simulink model "flightSimulation"  (R2026a)
settings: Solver=ode3  StartTime=0  StopTime=10  FixedStep=Ts  EnableMultiTasking=on
undefined symbols (not defined in the file or in its folder): ft, initPosSim3d, m, s, Ts
libraries: aerolibconvert2 x4, aerolibanimutils x2, environmentLibrary x2, sensorsLibrary x2, aerolibfltsims x2, aerolibsim3d x2, SignalEditorBlockLib x1, sim3dlib x1
settings Model: Creator=The MathWorks, Inc.  LastModifiedBy=The MathWorks, Inc.
settings OptimizationCC: BufferReuse=off
settings DebuggingCC: UnderspecifiedInitializationDetection=Classic  PregeneratedLibrarySubsystemCodeDiagnostic=none
settings HardwareCC: ProdHWDeviceType=32-bit Generic

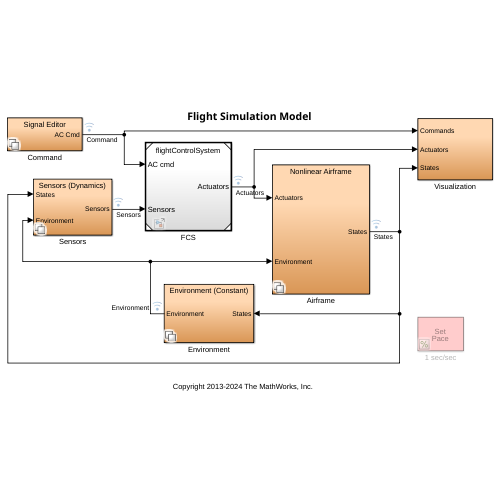
[thumbnail: Simulink's stored preview of the top-level diagram]
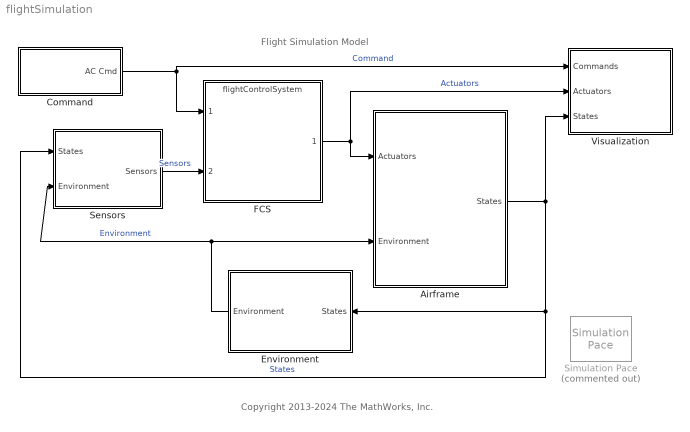
== system flightSimulation ==
  note: Flight Simulation Model
  note: Copyright 2013-2024 The MathWorks, Inc.
  Airframe : Subsystem  Variant=on
  Command : Subsystem  Variant=on
  Environment : Subsystem  Variant=on
  FCS : ModelReference  ModelNameDialog=flightControlSystem.slx  SimulationMode=Normal  ModelReferenceVersion=13.0
  Sensors : Subsystem  Variant=on
  Simulation Pace : aerolibanimutils/Simulation Pace  Commented=on  SimulationPace=1  SleepMode=MATLAB Thread  OutputPaceError=off  SampleTime=Ts
      settings: AttributesFormatString=%<SimulationPace> sec/sec
  Visualization : Subsystem
  wires:
  Command/1(AC Cmd) -> Visualization/1(Commands), FCS/1  "Command"
  Sensors/1(Sensors) -> FCS/2  "Sensors"
  FCS/1 -> Visualization/2(Actuators), Airframe/1(Actuators)  "Actuators"
  Environment/1(Environment) -> Sensors/2(Environment), Airframe/2(Environment)  "Environment"
  Airframe/1(States) -> Visualization/3(States), Environment/1(States), Sensors/1(States)  "States"

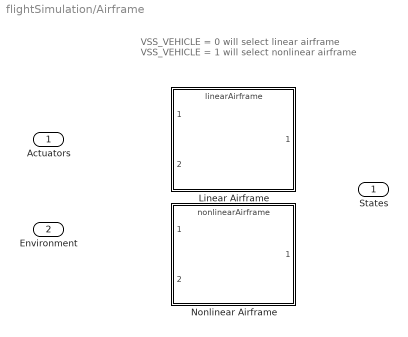
== system flightSimulation/Airframe ==
  note: VSS_VEHICLE = 0 will select linear airframe
      | VSS_VEHICLE = 1 will select nonlinear airframe
  Actuators : Inport
  Environment : Inport  Port=2  OutDataTypeStr=Bus: EnvironmentBus
  Linear Airframe : ModelReference  ModelNameDialog=linearAirframe.slx  SimulationMode=Normal  VariantControl=VSS_VEHICLE_LINEAR  ModelReferenceVersion=5.0
  Nonlinear Airframe : ModelReference  ModelNameDialog=nonlinearAirframe.slx  SimulationMode=Normal  VariantControl=VSS_VEHICLE_NONLINEAR  ModelReferenceVersion=13.0
  States : Outport  OutDataTypeStr=Bus: StatesBus  VectorParamsAs1DForOutWhenUnconnected=off

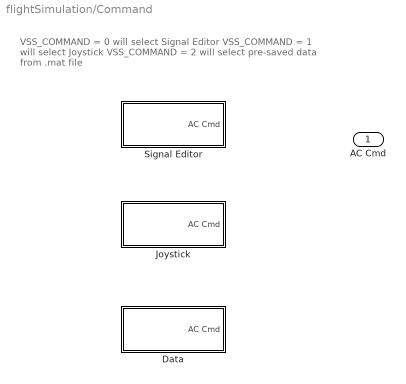
== system flightSimulation/Command ==
  note: VSS_COMMAND = 0 will select Signal Editor
      | VSS_COMMAND = 1 will select Joystick
      | VSS_COMMAND = 2 will select pre-saved data from .mat file
  Data : Subsystem  VariantControl=VSS_COMMAND_PRESAVED
  Joystick : Subsystem  VariantControl=VSS_COMMAND_JOYSTICK
  Signal Editor : Subsystem  VariantControl=VSS_COMMAND_SIGEDIT
  AC Cmd : Outport  OutDataTypeStr=Bus: CommandBus  VectorParamsAs1DForOutWhenUnconnected=off

== system flightSimulation/Environment ==
  note: VSS_ENVIRONMENT = 0 will select constant environment variables
      | VSS_ENVIRONMENT = 1 will select environment variables depending on position
  States : Inport  OutDataTypeStr=Bus: StatesBus
  Environment (Constant) : environmentLibrary/Environment (Constant)  SystemSampleTime=-1  VariantControl=VSS_ENVIRONMENT_CST  VariantActivationTime=update diagram  EmptyChoice=off  PassThrough=off  PassThroughVariantControl=(default)  EmptyChoiceVariantControl=(default)  AllowFlexibleInterface=on  Latency=0  AutoFrameSizeCalculation=off
  Environment (Variable) : environmentLibrary/Environment (Variable)  SystemSampleTime=-1  VariantControl=VSS_ENVIRONMENT_VARIABLE  VariantActivationTime=update diagram  EmptyChoice=off  PassThrough=off  PassThroughVariantControl=(default)  EmptyChoiceVariantControl=(default)  AllowFlexibleInterface=on  Latency=0  AutoFrameSizeCalculation=off
  Environment : Outport  OutDataTypeStr=Bus: EnvironmentBus  VectorParamsAs1DForOutWhenUnconnected=off

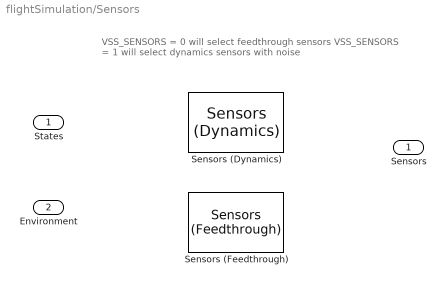
== system flightSimulation/Sensors ==
  note: VSS_SENSORS = 0 will select feedthrough sensors
      | VSS_SENSORS = 1 will select dynamics sensors with noise
  States : Inport
  Environment : Inport  Port=2
  Sensors (Dynamics) : sensorsLibrary/Sensors (Dynamics)  SystemSampleTime=-1  VariantControl=VSS_SENSORS_DYNAMICS  VariantActivationTime=update diagram  EmptyChoice=off  PassThrough=off  PassThroughVariantControl=(default)  EmptyChoiceVariantControl=(default)  AllowFlexibleInterface=on  Latency=0  AutoFrameSizeCalculation=off
  Sensors (Feedthrough) : sensorsLibrary/Sensors (Feedthrough)  SystemSampleTime=-1  VariantControl=VSS_SENSORS_FEEDTHROUGH  VariantActivationTime=update diagram  EmptyChoice=off  PassThrough=off  PassThroughVariantControl=(default)  EmptyChoiceVariantControl=(default)  AllowFlexibleInterface=on  Latency=0  AutoFrameSizeCalculation=off
  Sensors : Outport  VectorParamsAs1DForOutWhenUnconnected=off

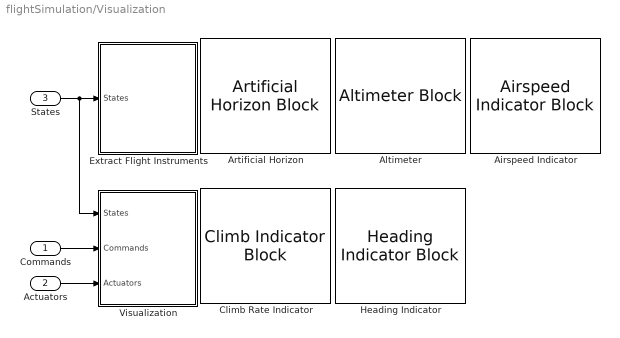
== system flightSimulation/Visualization ==
  Commands : Inport
  Actuators : Inport  Port=2
  States : Inport  Port=3
  Airspeed Indicator : AirspeedIndicatorBlock  LabelPosition=Hide  ScaleMin=0  ScaleMax=9
  Altimeter : AltimeterBlock  LabelPosition=Hide
  Artificial Horizon : ArtificialHorizonBlock  LabelPosition=Hide
  Climb Rate Indicator : ClimbIndicatorBlock  LabelPosition=Hide  ScaleMax=1000
  Extract Flight Instruments : Subsystem
  Heading Indicator : HeadingIndicatorBlock  LabelPosition=Hide
  Visualization : Subsystem  Variant=on
  wires:
  Commands/1 -> Visualization/2(Commands)
  States/1 -> Visualization/1(States), Extract Flight Instruments/1(States)
  Actuators/1 -> Visualization/3(Actuators)

== system flightSimulation/Command/Data ==
  Bus Creator : BusCreator  Inputs=4  OutDataTypeStr=Bus: CommandBus  NonVirtualBus=on
  Demux : Demux
  From File : FromFile  FileName=cmdData.mat  SampleTime=Ts
  AC Cmd : Outport  OutDataTypeStr=Bus: CommandBus  VectorParamsAs1DForOutWhenUnconnected=off
  wires:
  Bus Creator/1 -> AC Cmd/1
  Demux/1 -> Bus Creator/1  "roll_cmd"
  Demux/2 -> Bus Creator/2  "pitch_cmd"
  Demux/3 -> Bus Creator/3  "yaw_cmd"
  Demux/4 -> Bus Creator/4  "throttle_cmd"
  From File/1 -> Demux/1

== system flightSimulation/Command/Joystick ==
  Bus Creator : BusCreator  Inputs=4  OutDataTypeStr=Bus: CommandBus  NonVirtualBus=on
  Pilot Joystick : aerolibanimutils/Pilot Joystick  JoystickID=Joystick1  OutputConfiguration=FourAxis  SampleTime=Ts
  AC Cmd : Outport  OutDataTypeStr=Bus: CommandBus  VectorParamsAs1DForOutWhenUnconnected=off
  wires:
  Pilot Joystick/4 -> Bus Creator/4  "throttle_cmd"
  Pilot Joystick/3 -> Bus Creator/3  "yaw_cmd"
  Pilot Joystick/2 -> Bus Creator/2  "pitch_cmd"
  Pilot Joystick/1 -> Bus Creator/1  "roll_cmd"
  Bus Creator/1 -> AC Cmd/1

== system flightSimulation/Command/Signal Editor ==
  Signal Editor : SignalEditorBlockLib/Signal Editor  FileName=cmdSignalEditor.mat  ActiveScenario=Group1  ActiveSignal=CommandBus  IsBus=on  OutputBusObjectStr=Bus: CommandBus  SampleTime=0  Interpolate=off  ZeroCross=off  OutputAfterFinalValue=Setting to zero  Unit=inherit  PreserveSignalName=on  ApplySigPropsToAllScenarios=on  ApplySigPropsToAllSignals=off  SignalPropertySource=Dialog parameters
  AC Cmd : Outport  OutDataTypeStr=Bus: CommandBus  VectorParamsAs1DForOutWhenUnconnected=off
  wires:
  Signal Editor/1 -> AC Cmd/1

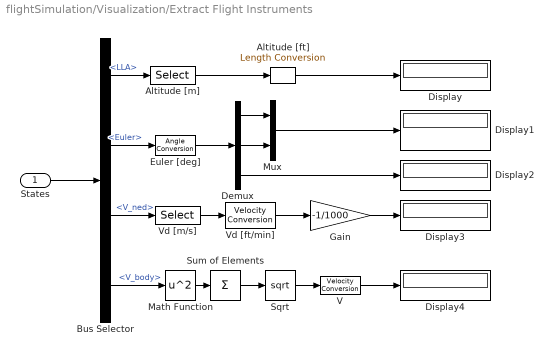
== system flightSimulation/Visualization/Extract Flight Instruments ==
  States : Inport
  Altitude [ft] : aerolibconvert2/Length Conversion  IU=m  OU=ft
  Altitude [m] : Selector  InputPortWidth=3  IndexOptions=Index vector (dialog)  Indices=[3]  OutputSizes=1
  Bus Selector : BusSelector  OutputSignals=LLA,Euler,V_ned,V_body
  Demux : Demux  Outputs=3
  Display{,1..4} (5 alike) : Display
  Euler [deg] : aerolibconvert2/Angle Conversion  IU=rad  OU=deg
  Gain : Gain  Gain=-1/1000
  Math Function : Math  Operator=square  SignedPower=on
  Mux : Mux  Inputs=2
  Sqrt : Sqrt
  Sum of Elements : Sum  Inputs=+
  V : aerolibconvert2/Velocity Conversion  IU=m/s  OU=kts
  Vd [ft/min] : aerolibconvert2/Velocity Conversion  IU=m/s  OU=ft/min
  Vd [m/s] : Selector  InputPortWidth=3  IndexOptions=Index vector (dialog)  Indices=[3]  OutputSizes=1
  wires:
  Bus Selector/1 -> Altitude [m]/1  "<LLA>"
  Altitude [m]/1 -> Altitude [ft]/1
  States/1 -> Bus Selector/1
  Altitude [ft]/1 -> Display/1
  Bus Selector/2 -> Euler [deg]/1  "<Euler>"
  Euler [deg]/1 -> Demux/1
  Demux/1 -> Mux/1
  Demux/2 -> Mux/2
  Mux/1 -> Display1/1
  Demux/3 -> Display2/1
  Bus Selector/3 -> Vd [m/s]/1  "<V_ned>"
  Vd [m/s]/1 -> Vd [ft/min]/1
  Vd [ft/min]/1 -> Gain/1
  Gain/1 -> Display3/1
  Math Function/1 -> Sum of Elements/1
  Sum of Elements/1 -> Sqrt/1
  Bus Selector/4 -> Math Function/1  "<V_body>"
  Sqrt/1 -> V/1
  V/1 -> Display4/1

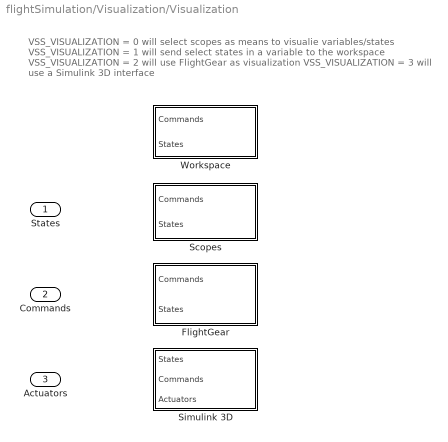
== system flightSimulation/Visualization/Visualization ==
  note: VSS_VISUALIZATION = 0 will select scopes as means to visualie variables/states
      | VSS_VISUALIZATION = 1 will send select states in a variable to the workspace
      | VSS_VISUALIZATION = 2 will use FlightGear as visualization
      | VSS_VISUALIZATION = 3 will use a Simulink 3D interface
  States : Inport  OutDataTypeStr=Bus: StatesBus
  Commands : Inport  Port=2  OutDataTypeStr=Bus: CommandBus
  Actuators : Inport  Port=3
  FlightGear : Subsystem  VariantControl=VSS_VISUALIZATION_FLIGHTGEAR
      mask init:
      | visualizationFlightGearVars;
  Scopes : Subsystem  VariantControl=VSS_VISUALIZATION_SCOPES
  Simulink 3D : Subsystem  VariantControl=VSS_VISUALIZATION_SL3D
      mask init:
      | visualizationFlightGearVars;
  Workspace : Subsystem  VariantControl=VSS_VISUALIZATION_WORKSPACE

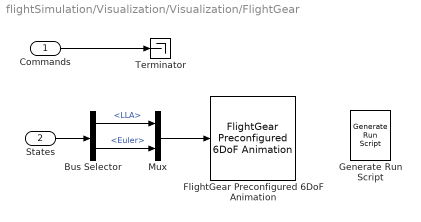
== system flightSimulation/Visualization/Visualization/FlightGear ==
  Commands : Inport
  States : Inport  Port=2
  Bus Selector : BusSelector  OutputSignals=LLA,Euler
  FlightGear Preconfigured 6DoF Animation : aerolibfltsims/FlightGear Preconfigured 6DoF Animation  xFlightGearVersion=v2017.3  DestinationIpAddress=Visualization.FlightGear.SixDOF.IPAddress  DestinationPort=Visualization.FlightGear.SixDOF.destinationPort  SampleTime=Ts  packetVersion=24
  Generate Run Script : aerolibfltsims/Generate Run Script  Architecture=Default  dataFlow=Send  GeometryModelName=Model  AirportId=KSFO  RunwayId=10L  InitialAltitude=Visualization.FlightGear.generateRunScript.initialAltitude  InitialHeading=Visualization.FlightGear.generateRunScript.initialHeading  OffsetDistance=Visualization.FlightGear.generateRunScript.offsetDistance  OffsetAzimuth=Visualization.FlightGear.generateRunScript.offsetAzimuth  InstallScenery=off  DisableShaders=off  OriginAddress=127.0.0.1  DestinationPort=Visualization.FlightGear.generateRunScript.destinationPort  OriginPort=5505  LocalAddress=127.0.0.1  OutputFileName=runfg.bat  FlightGearBaseDirectory=C:\Program Files\FlightGear
  Mux : Mux  Inputs=2
  Terminator : Terminator
  wires:
  States/1 -> Bus Selector/1
  Bus Selector/1 -> Mux/1  "<LLA>"
  Bus Selector/2 -> Mux/2  "<Euler>"
  Mux/1 -> FlightGear Preconfigured 6DoF Animation/1
  Commands/1 -> Terminator/1

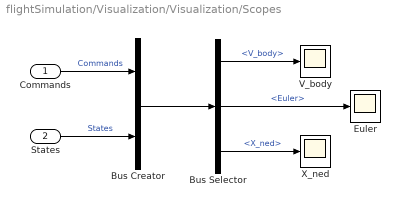
== system flightSimulation/Visualization/Visualization/Scopes ==
  Commands : Inport
  States : Inport  Port=2
  Bus Creator : BusCreator  Inputs=2
  Bus Selector : BusSelector  OutputSignals=States.V_body,States.Euler,States.X_ned
  Euler : Scope
      settings: ActiveDisplayYMinimum=-0.0140044  ActiveDisplayYMaximum=0.125876  DataLoggingVariableName=ScopeData2
  V_body : Scope
      settings: ActiveDisplayYMinimum=-2.96824  ActiveDisplayYMaximum=14.7064
  X_ned : Scope
      settings: ActiveDisplayYMinimum=-0.0140044  ActiveDisplayYMaximum=0.125876
  wires:
  Commands/1 -> Bus Creator/1  "Commands"
  States/1 -> Bus Creator/2  "States"
  Bus Creator/1 -> Bus Selector/1
  Bus Selector/1 -> V_body/1  "<V_body>"
  Bus Selector/2 -> Euler/1  "<Euler>"
  Bus Selector/3 -> X_ned/1  "<X_ned>"

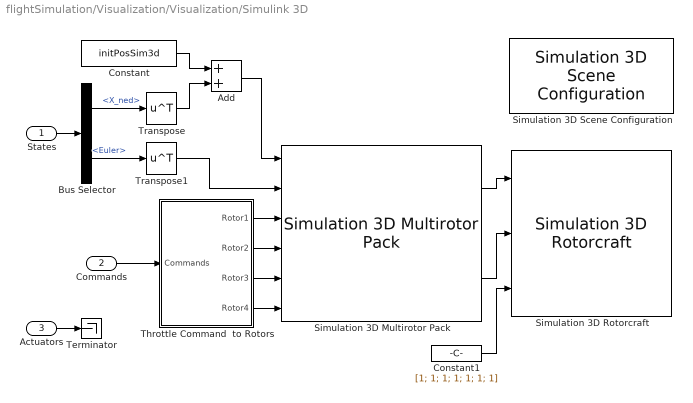
== system flightSimulation/Visualization/Visualization/Simulink 3D ==
  States : Inport
  Commands : Inport  Port=2
  Actuators : Inport  Port=3
  Add : Sum
  Bus Selector : BusSelector  OutputSignals=X_ned,Euler
  Constant : Constant  Value=initPosSim3d  VectorParams1D=off
  Constant1 : Constant  Value=[1; 1; 1; 1; 1; 1; 1]  VectorParams1D=off
  Simulation 3D Multirotor Pack : aerolibsim3d/Simulation 3D Multirotor Pack  Rotor1_T=off  Rotor1_R=on  Rotor2_T=off  Rotor2_R=on  Rotor3_T=off  Rotor3_R=on  Rotor4_T=off  Rotor4_R=on  Rotor5_T=off  Rotor5_R=off  Rotor6_T=off  Rotor6_R=off  Rotor7_T=off  Rotor7_R=off  Rotor8_T=off  Rotor8_R=off  Sensor1_T=off  Sensor1_R=off  Sensor2_T=off  Sensor2_R=off  EnableUETransform=on  GeoRadioButton=NED
      settings: AttributesFormatString=NED
  Simulation 3D Rotorcraft : aerolibsim3d/Simulation 3D Rotorcraft  Priority=-1  Mesh=Multirotor  MeshPath=/MathWorksAerospaceContent/Vehicles/Rotorcraft/Helicopter/Mesh/SK_Helicopter.SK_Helicopter  MeshPathLight=/MathWorksAerospaceContent/Vehicles/Rotorcraft/LightHelicopter/Mesh/SK_LightHelicopter.SK_LightHelicopter  MeshPathMulti=/MathWorksAerospaceContent/Vehicles/Rotorcraft/Multirotor/Mesh/SK_Quadcopter.SK_Quadcopter  AircraftColor=Red  ActorName=Sim3dQuadcopter  Translation=[initPosSim3d; zeros(10,3)]  Rotation=zeros(11,3)  ScaleInputPort=Dialog  Scale=[1 1 1]  InitialScale=[1 1 1]  IsGHSensorEnabled=off  AreGHRaysVisible=off  IsOutputReshapeEnabled=off  GHRayLength=1524  GHBodyOffset=1.169  GHFrontTireRadius=0.196  GHLeftTireRadius=0.203  GHRightTireRadius=0.203  GHContactLocation1=[1.47 -1.04 1.169]  GHContactLocation2=[-1.24 -1.04 1.169]  GHContactLocation3=[-1.24 1.04 1.169]  GHContactLocation4=[1.47 1.04 1.169]  WoWSensorTolerance=0.05  LightsConfig=Configurable lights  LandingLightIntensity=300000  LandingLightConeAngle=15  LandingLightColor=[1 1 1]  HelicopterLeftLandingLightLocation=[0 0 0]  HelicopterLeftLandingLightOrientation=[0 0 0]  NoseLightIntensity=150000  NoseLightConeAngle=36  HelicopterNoseLightLocation=[0 0 0]  HelicopterNoseLightOrientation=[0 0 0]  NavLightIntensity=500  PositionLightIntensity=500  StrobeLightIntensity=5000  StrobeLightColor=[1 1 1]  StrobePeriod=2  StrobePulseWidth=10  BeaconLightIntensity=4000  BeaconLightColor=[1 0 0]  BeaconPeriod=2  BeaconPulseWidth=10  SampleTime=-1  ActorType=SimulinkVehicle  ID=C  aMode=0  ActorTag=Sim3dQuadcopter
  Simulation 3D Scene Configuration : sim3dlib/Simulation 3D Scene Configuration  Priority=0  ProjectFormat=Default Scenes  SceneDesc=Airport  ProjectName=/mathworks/devel/bat/filer/batfs2553-0/BR2026ad.3276743.BR2026ad.3269917.pass/build/matlab/toolbox/shared/sim3d_projects/automotive_project_linux/UE/LinuxNoEditor/VehicleSimulation.sh  ScenePath=/Game/Maps/HwStrght  EnableOpenDRIVE=off  vehTagList={'Custom';'Scene Origin';'Sim3dQuadcopter'}  vehTag=Sim3dQuadcopter  AttachedCameraRelativeTranslation=[0 0 0]  FreeCameraDefaultInitialTranslation=[-6, 0, 2]  AttachedCameraRelativeRotation=[0, -15, 0]  FreeCameraDefaultInitialRotation=[0, -15, 0]  ViewpointName=Custom  FreeCameraInitialTranslation=[-6, 0, 2]  FreeCameraInitialRotation=[0, -15, 0]  OpVisEn=off  Ts=Ts  EnableWindow=on  EnableRemoteAccess=off  SimulationMode=CoSimulation  SimulateUsing=Interpreted execution  EnableAnimationRecording=off  OverrideDefaultRecording=off  AnimationRecordingFileName=sim3dAnimation.mat  AnimationRecordingInterval=[0 inf]  EnableWeather=off  SunAzimuth=90  SunAltitude=40.0  EnableGeospatialSun=off  Latitude=0  Longitude=0  Date=2023-01-01  Time=10:30:00  GeoTimeZone=-5.0  SunDaylightSaving=off  wind=1  clouds=10  EnableVolumetricClouds=off  CloudCoverage=0  CloudAltitude=6  fog=0  rain=0  RaindropsEffect=off  SnowDensity=0  EnableGeospatial=off  TilesetSource=Earth terrain  UseTrueOrigin=off  OriginHeight=200  OriginLatitude=40.744652  OriginLongitude=-73.988864  MapStyle=Aerial  AdditionalAssetIDs=[]  UseAdvancedSunSky=off  SolarTime=11  TimeZone=-5  Day=21  Month=9  Year=2022  UseDaylightSavingTime=on  DSTStartDay=10  DSTStartMonth=3  DSTEndDay=3  DSTEndMonth=11  DSTSwitchHour=2  sensorTag=MainCamera1  sensorId=1  sensorName=MainCamera1  mountLoc=Origin  offsetFlag=off  tmountOffset=[0, 0, 0]  rmountOffset=[0, 0, 0]  HorizontalResolution=1280  VerticalResolution=720  HorizontalFOV=60  mountPoint=[0 0 0]  mountOrientation=[0 0 0]  aMode=0  ID=1  GeoTrigger=Inactive  ViewNameList={'Custom'}  ViewTranslationList={'[-6 0 2]'}  ViewRotationList={'[0 -15 0]'}
      settings: AttributesFormatString=NED  LibrarySourceBlock=aerolibsim3d/Simulation 3D Scene Configuration
  Terminator : Terminator
  Throttle Command  to Rotors : Subsystem
  Transpose : Math  Operator=transpose
  Transpose1 : Math  Operator=transpose
  wires:
  States/1 -> Bus Selector/1
  Throttle Command  to Rotors/1(Rotor1) -> Simulation 3D Multirotor Pack/3
  Throttle Command  to Rotors/2(Rotor2) -> Simulation 3D Multirotor Pack/4
  Throttle Command  to Rotors/3(Rotor3) -> Simulation 3D Multirotor Pack/5
  Throttle Command  to Rotors/4(Rotor4) -> Simulation 3D Multirotor Pack/6
  Constant/1 -> Add/1
  Add/1 -> Simulation 3D Multirotor Pack/1
  Bus Selector/1 -> Transpose/1  "<X_ned>"
  Transpose/1 -> Add/2
  Bus Selector/2 -> Transpose1/1  "<Euler>"
  Transpose1/1 -> Simulation 3D Multirotor Pack/2
  Simulation 3D Multirotor Pack/1 -> Simulation 3D Rotorcraft/1
  Simulation 3D Multirotor Pack/2 -> Simulation 3D Rotorcraft/2
  Constant1/1 -> Simulation 3D Rotorcraft/3
  Actuators/1 -> Terminator/1
  Commands/1 -> Throttle Command  to Rotors/1(Commands)

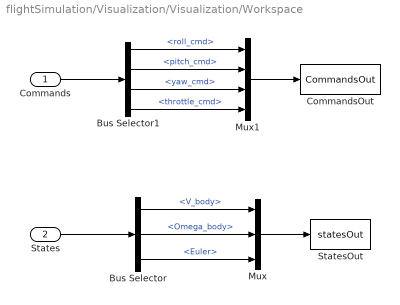
== system flightSimulation/Visualization/Visualization/Workspace ==
  Commands : Inport
  States : Inport  Port=2
  Bus Selector : BusSelector  OutputSignals=V_body,Omega_body,Euler
  Bus Selector1 : BusSelector  OutputSignals=roll_cmd,pitch_cmd,yaw_cmd,throttle_cmd
  CommandsOut : ToWorkspace  VariableName=CommandsOut  SaveFormat=Structure With Time  SampleTime=-1
  Mux : Mux  Inputs=3
  Mux1 : Mux
  StatesOut : ToWorkspace  VariableName=statesOut  SaveFormat=Structure With Time  SampleTime=-1
  wires:
  States/1 -> Bus Selector/1
  Bus Selector/2 -> Mux/2  "<Omega_body>"
  Bus Selector/3 -> Mux/3  "<Euler>"
  Bus Selector/1 -> Mux/1  "<V_body>"
  Mux/1 -> StatesOut/1
  Commands/1 -> Bus Selector1/1
  Bus Selector1/2 -> Mux1/2  "<pitch_cmd>"
  Bus Selector1/1 -> Mux1/1  "<roll_cmd>"
  Mux1/1 -> CommandsOut/1
  Bus Selector1/4 -> Mux1/4  "<throttle_cmd>"
  Bus Selector1/3 -> Mux1/3  "<yaw_cmd>"

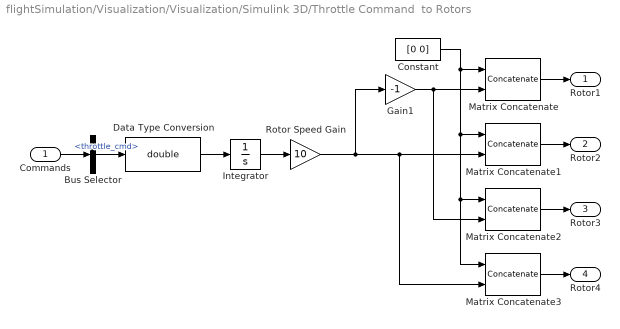
== system flightSimulation/Visualization/Visualization/Simulink 3D/Throttle Command  to Rotors ==
  Commands : Inport
  Bus Selector : BusSelector  OutputSignals=throttle_cmd
  Constant : Constant  Value=[0 0]  VectorParams1D=off
  Data Type Conversion : DataTypeConversion  OutDataTypeStr=double  SaturateOnIntegerOverflow=off  RndMeth=Floor
  Gain1 : Gain  Gain=-1
  Integrator : Integrator
  Matrix Concatenate{,1..3} (4 alike) : Concatenate  Mode=Multidimensional array  ConcatenateDimension=2
  Rotor Speed Gain : Gain  Gain=10
  Rotor1 : Outport
  Rotor2 : Outport  Port=2
  Rotor3 : Outport  Port=3
  Rotor4 : Outport  Port=4
  wires:
  Matrix Concatenate/1 -> Rotor1/1
  Matrix Concatenate3/1 -> Rotor4/1
  Matrix Concatenate2/1 -> Rotor3/1
  Matrix Concatenate1/1 -> Rotor2/1
  Constant/1 -> Matrix Concatenate3/1, Matrix Concatenate2/1, Matrix Concatenate1/1, Matrix Concatenate/1
  Commands/1 -> Bus Selector/1
  Bus Selector/1 -> Data Type Conversion/1  "<throttle_cmd>"
  Data Type Conversion/1 -> Integrator/1
  Integrator/1 -> Rotor Speed Gain/1
  Gain1/1 -> Matrix Concatenate2/2, Matrix Concatenate/2
  Rotor Speed Gain/1 -> Gain1/1, Matrix Concatenate3/2, Matrix Concatenate1/2
